simulink model "ClarkePark"  (R2026b)
settings: Solver=VariableStepAuto
PostLoadFcn:
  | mathSrc=fileparts(get_param(bdroot,'FileName'));addpath(fullfile(mathSrc,'clarke'),fullfile(mathSrc,'park'));clear mathSrc;
libraries: ClarkeTransforms x2, ParkTransforms x2
settings Model: Creator=24322  LastModifiedBy=24322

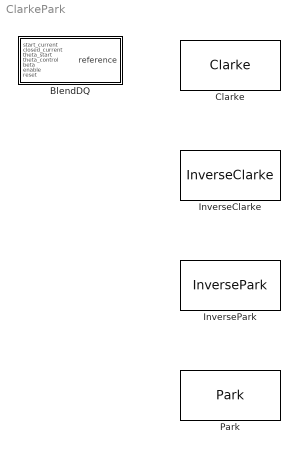
== system ClarkePark ==
  BlendDQ : Subsystem
  Clarke : ClarkeTransforms/Clarke  SystemSampleTime=-1  VariantActivationTime=update diagram  EmptyChoice=off  PassThrough=off  PassThroughVariantControl=(default)  EmptyChoiceVariantControl=(default)  AllowFlexibleInterface=on  Latency=0  AutoFrameSizeCalculation=off
  InverseClarke : ClarkeTransforms/InverseClarke  SystemSampleTime=-1  VariantActivationTime=update diagram  EmptyChoice=off  PassThrough=off  PassThroughVariantControl=(default)  EmptyChoiceVariantControl=(default)  AllowFlexibleInterface=on  Latency=0  AutoFrameSizeCalculation=off
  InversePark : ParkTransforms/InversePark  SystemSampleTime=-1  VariantActivationTime=update diagram  EmptyChoice=off  PassThrough=off  PassThroughVariantControl=(default)  EmptyChoiceVariantControl=(default)  AllowFlexibleInterface=on  Latency=0  AutoFrameSizeCalculation=off
  Park : ParkTransforms/Park  SystemSampleTime=-1  VariantActivationTime=update diagram  EmptyChoice=off  PassThrough=off  PassThroughVariantControl=(default)  EmptyChoiceVariantControl=(default)  AllowFlexibleInterface=on  Latency=0  AutoFrameSizeCalculation=off

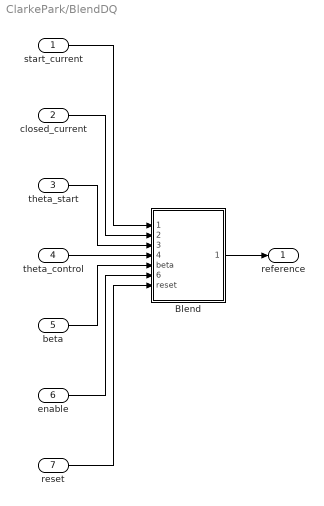
== system ClarkePark/BlendDQ ==
  start_current : Inport
  closed_current : Inport  Port=2
  theta_start : Inport  Port=3
  theta_control : Inport  Port=4
  beta : Inport  Port=5
  enable : Inport  Port=6
  reset : Inport  Port=7
  Blend : MATLAB Function  TreatAsAtomicUnit=on
  reference : Outport
  wires:
  Blend/1(reference) -> reference/1
  reset/1 -> Blend/7(reset)
  enable/1 -> Blend/6(enable)
  beta/1 -> Blend/5(beta)
  theta_control/1 -> Blend/4(thetaControl)
  theta_start/1 -> Blend/3(thetaStart)
  closed_current/1 -> Blend/2(closedCurrent)
  start_current/1 -> Blend/1(startCurrent)

== matlab function ClarkePark/BlendDQ/Blend ==
  data: startCurrent input; reference output; closedCurrent input; thetaStart input; thetaControl input; beta input; enable input; reset input
function reference=blend_dq(startCurrent,closedCurrent,thetaStart,thetaControl,beta,enable,reset)
%#codegen
%BLEND_DQ Mix two current references after transforming to a common frame.
reference=zeros(2,1,'like',startCurrent);
if enable<0.5 || reset>0.5,return,end
delta=cast(thetaStart-thetaControl,'like',startCurrent);
fraction=min(max(cast(beta,'like',startCurrent),0),1);
rotation=[cos(delta),-sin(delta);sin(delta),cos(delta)];
start=[startCurrent(1);startCurrent(2)];
closed=cast([closedCurrent(1);closedCurrent(2)],'like',startCurrent);
reference=(1-fraction)*(rotation*start)+fraction*closed;
end
